simulink model "MIL2"  (R2024b)
settings: Solver=VariableStepAuto  StartTime=0.0  StopTime=0.4  RelTol=1e-3
InitFcn:
  | load('Khinf_QBC_MIL2.mat')
values from neighbouring files (symbols this model uses):
  Ak2 = [0.99999000005 -0.874071604568 92.4139805098 83.0101069502 -184.481272036 -40.5453136884 4.23629025743e-17 -0.390736622587 -19.8991754296 -17.8742726102 39.723699547 8.73047893275 ... (36 elements, 6x6)]    [Khinf_QBC_MIL2.mat]    (also in hinf_discretize_MIL2.m = Kd2.A)
  Bk2 = [0.00079999600002 -0.000349628641827 0.0369655922039 0.0332040427801 -0.0737925088144 -0.0162181254754]    [Khinf_QBC_MIL2.mat]    (also in hinf_discretize_MIL2.m = Kd2.B)
  Ck2 = [17.170141268 -3.69718576515 -0.619129874971 -0.385866142002 -0.162165465963 -0.570961814906]    [Khinf_QBC_MIL2.mat]    (also in hinf_discretize_MIL2.m = Kd2.C)
  Dk2 = 0.00686805650718    [Khinf_QBC_MIL2.mat]    (also in hinf_discretize_MIL2.m = Kd2.D)
  t_vin = 0.2    [mil_metrics2_vin.m]
  Ts2 = 0.0001    [Khinf_QBC_MIL2.mat]    (also in hinf_discretize_MIL2.m = 1/fs)
  Vin_nom = 18    [mil_metrics2_vin.m]
  Vin_step = Vin_nom*(1+vin_pct)    (= 16.2)    [mil_metrics2_vin.m]
undefined symbols (not defined in the file or in its folder): controller_init, D0, dend, DiscIntNeverNeededParam, dspblkCoreblockFVToolHelper, eta, gcbh, Iint_max, K_smc, Ki, Kx, lambda1, numd, phi, Rnom, Tc, Vin, x_op, xi_max
libraries: spsSeriesRLCBranchLib x5, spsCurrentMeasurementLib x3, spsDiodeLib x3, spsVoltageMeasurementLib x3, spsMeanLib x2, spsControlledVoltageSourceLib x1, spsDCVoltageSourceLib x1, slpidlib x1, spsGroundLib x1, spsMosfetLib x1, spsPWMGeneratorDCDCLib x1, sps_lib x1
settings Model: Creator=Asus  LastModifiedBy=yohan
settings ConfigComp: CovMetricSettings=de

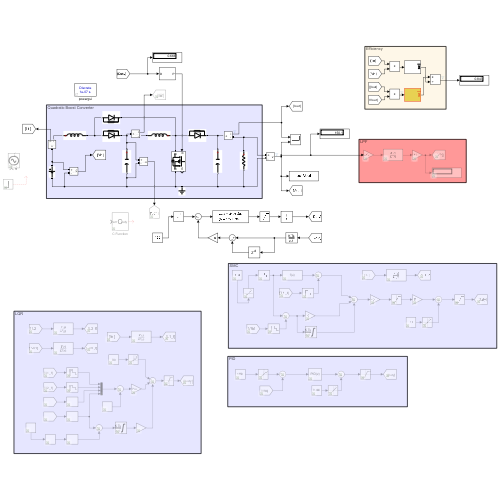
[thumbnail: Simulink's stored preview of the top-level diagram]
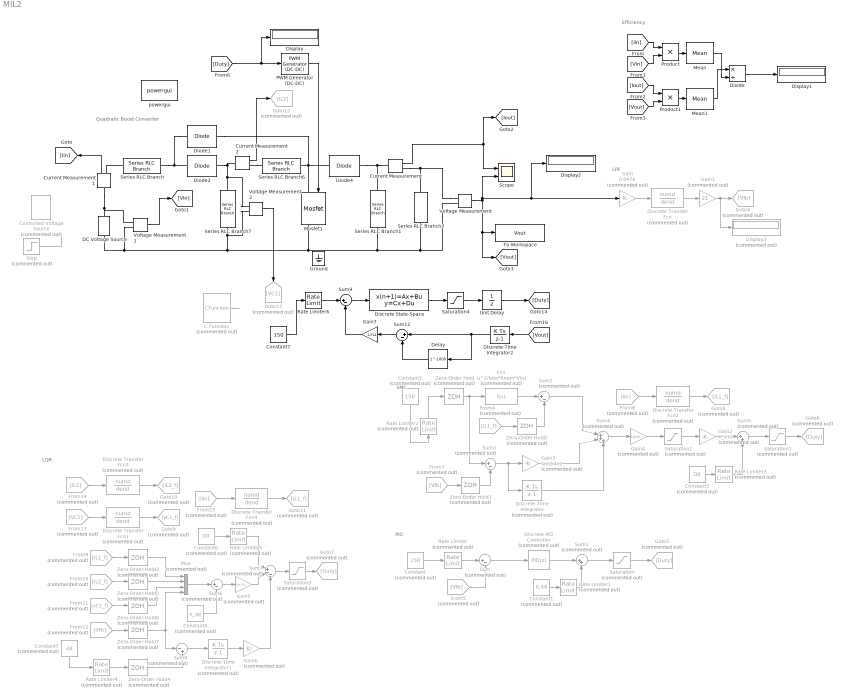
== system MIL2 ==
  note: SMC
  note: LQR
  note: PID
  note: Efficiency
  note: Quadratic Boost Converter
  note: LPF
  C Function : CFunction  Commented=on  OutputCode=duty = controller_step(err, 0.0f);  StartCode=controller_init();  CodegenOutputCode=duty = controller_step(err, 0.0f);  CodegenStartCode=controller_init();  SimCustomHeaderFile=controller_step.h  SimCustomSourceFile=controller_step.c  CustomHeaderFile=controller_step.h  CustomSourceFile=controller_step.c
  Constant : Constant  Commented=on  Value=150
  Constant1 : Constant  Commented=on  Value=0.44
  Constant2 : Constant  Commented=on  Value=150
  Constant3 : Constant  Commented=on  Value=D0
  Constant4 : Constant  Commented=on  Value=x_op
  Constant5 : Constant  Commented=on  Value=48
  Constant6 : Constant  Commented=on  Value=D0
  Constant7 : Constant  Value=150
  Controlled Voltage Source : spsControlledVoltageSourceLib/Controlled Voltage Source  Commented=on  Initialize=on  Source_Type=DC  Amplitude=18  Phase=0  Frequency=0  Measurements=None
  Current Measurement : spsCurrentMeasurementLib/Current Measurement  PhasorSimulation=off  OutputType=Complex  PSBequivalent=0
  Current Measurement1 : spsCurrentMeasurementLib/Current Measurement  PhasorSimulation=off  OutputType=Complex  PSBequivalent=0
  Current Measurement2 : spsCurrentMeasurementLib/Current Measurement  PhasorSimulation=off  OutputType=Complex  PSBequivalent=0
  DC Voltage Source : spsDCVoltageSourceLib/DC Voltage Source  Amplitude=18  Measurements=None
  Delay : Delay  DelayLength=1000  InitialCondition=0  SampleTime=1e-7
  Diode1 : spsDiodeLib/Diode  Ron=0.001  Lon=0  Vf=0  IC=0  UseSnubber=off  Rs=500  Cs=250e-9  Measurements=off
  Diode2 : spsDiodeLib/Diode  Ron=0.001  Lon=0  Vf=0  IC=0  UseSnubber=off  Rs=500  Cs=250e-9  Measurements=off
  Diode4 : spsDiodeLib/Diode  Ron=0.001  Lon=0  Vf=0.8  IC=0  UseSnubber=off  Rs=500  Cs=250e-9  Measurements=off
  Discrete Transfer Fcn{,1..4} (5 alike) : DiscreteTransferFcn  Commented=on  LoadFcn=dspblkCoreblockFVToolHelper(gcbh,'load');  Numerator=numd  Denominator=dend
      settings: CopyFcn=dspblkCoreblockFVToolHelper(gcbh,'copy');  DeleteFcn=dspblkCoreblockFVToolHelper(gcbh,'close');  ModelCloseFcn=dspblkCoreblockFVToolHelper(gcbh,'close');  PreSaveFcn=dspblkCoreblockFVToolHelper(gcbh,'presave');  PostSaveFcn=dspblkCoreblockFVToolHelper(gcbh,'postsave');  CloseFcn=dspblkCoreblockFVToolHelper(gcbh,'close');
  Discrete PID Controller : slpidlib/PID Controller  Commented=on  Controller=PID  Form=Parallel  TimeDomain=Discrete-time  UseExternalTs=off  SampleTime=2e-5  IntegratorMethod=Forward Euler  FilterMethod=Forward Euler  ControllerParametersSource=internal  P=1.0407e-3  I=2.0814e-2  UseKiTs=off  D=2.0814e-6  UseExternalDerivativeSource=off  N=100  UseFilter=on  TunerSelectOption=Transfer Function Based (PID Tuner App)  InitialConditionSource=internal  InitialConditionForIntegrator=0  InitialConditionForFilter=0  DifferentiatorICPrevScaledInput=0  ExternalReset=none  TrackingMode=off  Kt=1  LimitOutput=off  SatLimitsSource=internal  UpperSaturationLimit=inf  LowerSaturationLimit=-inf  LinearizeAsGain=off  AntiWindupMode=none  Kb=1  LimitIntegrator=off  UpperIntegratorSaturationLimit=inf  LowerIntegratorSaturationLimit=-inf  POutMin=[]  POutMax=[]  IOutMin=[]  IOutMax=[]  DOutMin=[]  DOutMax=[]  NOutMin=[]  NOutMax=[]  SumOutMin=[]  SumOutMax=[]  SaturationOutMin=[]  SaturationOutMax=[]  PParamMin=[]  PParamMax=[]  IParamMin=[]  IParamMax=[]  DParamMin=[]  DParamMax=[]  NParamMin=[]  NParamMax=[]  KbParamMin=[]  KbParamMax=[]  KtParamMin=[]  KtParamMax=[]  KbOutMin=[]  KbOutMax=[]  KtOutMin=[]  KtOutMax=[]  IntegratorOutMin=[]  IntegratorOutMax=[]  FilterOutMin=[]  FilterOutMax=[]  SumI1OutMin=[]  SumI1OutMax=[]  SumI2OutMin=[]  SumI2OutMax=[]  SumI3OutMin=[]  SumI3OutMax=[]  SumI4OutMin=[]  SumI4OutMax=[]  SumDOutMin=[]  SumDOutMax=[]  DifferentiatorOutMin=[]  DifferentiatorOutMax=[]  FilterDiffOutCoefMin=[]  FilterDiffOutCoefMax=[]  ReciprocalOutMin=[]  ReciprocalOutMax=[]  SumDenOutMin=[]  SumDenOutMax=[]  SumNumOutMin=[]  SumNumOutMax=[]  DivideOutMin=[]  DivideOutMax=[]  UdiffTsProdOutMin=[]  UdiffTsProdOutMax=[]  NTsProdOutMin=[]  NTsProdOutMax=[]  UintegralTsProdOutMin=[]  UintegralTsProdOutMax=[]  UngainTsProdOutMin=[]  UngainTsProdOutMax=[]  ClampingZeroOutDataTypeStr=Inherit: Inherit via back propagation  ClampingZeroOutMin=[]  ClampingZeroOutMax=[]  FilterDenConstantOutDataTypeStr=Inherit: Inherit via back propagation  FilterDenConstantOutMin=[]  FilterDenConstantOutMax=[]  PCopyOutDataTypeStr=Inherit: Inherit via back propagation  PCopyOutMin=[]  PCopyOutMax=[]  NCopyOutDataTypeStr=Inherit: Inherit via back propagation  NCopyOutMin=[]  NCopyOutMax=[]  IntegratorContinuousStateAttributes=''  IntegratorStateMustResolveToSignalObject=off  IntegratorRTWStateStorageClass=Auto  FilterContinuousStateAttributes=''  FilterStateMustResolveToSignalObject=off  FilterRTWStateStorageClass=Auto  ParallelPVariant=InternalParameters  IdealPVariant=Disabled  IVariant=InternalParameters  DVariant=InternalParameters  IntegratorVariant=Discrete  SatVariant=Disabled  AWVariant=Passthrough  PCopyVariant=Disabled  TRVariant=Disabled  FdbkBlocksVariant=Forward  IdealPFdbkVariant=Disabled  SatFdbkVariant=Disabled  DerivativeFilterVariant=ForwardEulerFilter  NVariant=InternalParameters  NCopyVariant=Disabled  FilterICVariant=InternalICsFilter  IntegratorICVariant=InternalICs  ExternalResetVariant=Disabled  TRSumVariant=Passthrough  SumFdbkVariant=Disabled  SumVariant=Sum_PID  TsampFilterVariant=InternalTs  TsampNgainVariant=Passthrough  TsampIntegralVariant=Disabled_SignalSpec  ExternalSaturationOutDataTypeStr=Inherit: Same as second input  DerivativeSourceVariant=ErrorSignal  PreIntVariant=InternalPreInt
      settings: LibrarySourceBlock=simulink/Discrete/Discrete PID Controller
  Discrete State-Space : DiscreteStateSpace  A=Ak2  B=Bk2  C=Ck2  D=Dk2  SampleTime=Ts2
  Discrete-Time Integrator : DiscreteIntegrator  Commented=on  gainval=lambda2  SampleTime=Tc  LimitOutput=on  UpperSaturationLimit=Iint_max  LowerSaturationLimit=-Iint_max  ICPrevOutput=DiscIntNeverNeededParam  ICPrevScaledInput=DiscIntNeverNeededParam
  Discrete-Time Integrator1 : DiscreteIntegrator  Commented=on  SampleTime=Tc  LimitOutput=on  UpperSaturationLimit=xi_max  LowerSaturationLimit=-xi_max  ICPrevOutput=DiscIntNeverNeededParam  ICPrevScaledInput=DiscIntNeverNeededParam
  Discrete-Time Integrator2 : DiscreteIntegrator  SampleTime=1e-7  ICPrevOutput=DiscIntNeverNeededParam  ICPrevScaledInput=DiscIntNeverNeededParam
  Display : Display
  Display1 : Display
  Display2 : Display
  Display3 : Display  Commented=on
  Divide : Product  Inputs=*/
  Fcn : Fcn  Commented=on  Expr=u^2/(eta*Rnom*Vin)
  From10 : From  Commented=on  GotoTag=iL2_f
  From11 : From  Commented=on  GotoTag=vC1_f
  From12 : From  Commented=on  GotoTag=Vfb
  From13 : From  Commented=on  GotoTag=VC1
  From14 : From  Commented=on  GotoTag=IL2
  From15 : From  Commented=on  GotoTag=Iin
  From4 : From  Commented=on  GotoTag=iL1_f
  From5 : From  Commented=on  GotoTag=Vfb
  From7 : From  Commented=on  GotoTag=Vfb
  From8 : From  Commented=on  GotoTag=Iin
  From9 : From  Commented=on  GotoTag=iL1_f
  Gain : Gain  Commented=on  Gain=0.0476
  Gain1 : Gain  Commented=on  Gain=21
  Gain2 : Gain  Commented=on  Gain=K_smc
  Gain3 : Gain  Commented=on  Gain=lambda1
  Gain4 : Gain  Commented=on  Gain=1/phi
  Gain5 : Gain  Commented=on  Gain=Kx  Multiplication=Matrix(K*u)
  Gain6 : Gain  Commented=on  Gain=Ki
  Gain7 : Gain  Gain=1/Ts2
  Goto10 : Goto  Commented=on  GotoTag=iL2_f
  Goto11 : Goto  Commented=on  GotoTag=iL1_f
  Goto12 : Goto  Commented=on  GotoTag=IL2
  Goto13 : Goto  Commented=on  GotoTag=VC1
  Goto4 : Goto  Commented=on  GotoTag=Vfb
  Goto5 : Goto  Commented=on  GotoTag=Duty
  Goto6 : Goto  Commented=on  GotoTag=Duty
  Goto7 : Goto  Commented=on  GotoTag=Duty
  Goto8 : Goto  Commented=on  GotoTag=iL1_f
  Goto9 : Goto  Commented=on  GotoTag=vC1_f
  Ground : spsGroundLib/Ground  LConnTagsString=a
  Mean : spsMeanLib/Mean  Freq=1000  Vinit=0  Ts=0
  Mean1 : spsMeanLib/Mean  Freq=1000  Vinit=0  Ts=0
  Mosfet1 : spsMosfetLib/Mosfet  Ron=0.1  Lon=0  Rd=0.01  Vfd=0  IC=0  Rs=1e5  Cs=inf  Measurements=on
  Mux : Mux  Commented=on
  PWM Generator (DC-DC) : spsPWMGeneratorDCDCLib/PWM Generator (DC-DC)  Fsw=10000  Ts=0
  Product : Product
  Product1 : Product
  Rate Limiter : RateLimiter  Commented=on  RisingSlewLimit=1600  SampleTimeMode=inherited
  Rate Limiter1 : RateLimiter  Commented=on  RisingSlewLimit=15  SampleTimeMode=inherited
  Rate Limiter2 : RateLimiter  Commented=on  RisingSlewLimit=1600  FallingSlewLimit=-inf  SampleTimeMode=inherited
  Rate Limiter3 : RateLimiter  Commented=on  RisingSlewLimit=15  FallingSlewLimit=-inf  SampleTimeMode=inherited
  Rate Limiter4 : RateLimiter  Commented=on  RisingSlewLimit=1600  FallingSlewLimit=-inf  SampleTimeMode=inherited
  Rate Limiter5 : RateLimiter  Commented=on  RisingSlewLimit=15  FallingSlewLimit=-inf  SampleTimeMode=inherited
  Rate Limiter6 : RateLimiter  RisingSlewLimit=150/0.025  FallingSlewLimit=-150/0.025  SampleTimeMode=inherited
  Saturation : Saturate  Commented=on  UpperLimit=0.8  LowerLimit=0
  Saturation1 : Saturate  Commented=on  UpperLimit=0.6  LowerLimit=0
  Saturation2 : Saturate  Commented=on  UpperLimit=1  LowerLimit=-1
  Saturation3 : Saturate  Commented=on  UpperLimit=0.6  LowerLimit=0
  Saturation4 : Saturate  UpperLimit=5  LowerLimit=-5
  Scope : Scope  NumInputPorts=2
      settings: InitFcn=load('Khinf_QBC_MIL1.mat')  OpenFcn=load('Khinf_QBC_MIL1.mat')
  Series RLC Branch : spsSeriesRLCBranchLib/Series RLC Branch  LConnTagsString=__new0  RConnTagsString=__new0  BranchType=L  Resistance=0.005  Inductance=0.001  SetiL0=off  InitialCurrent=0  Capacitance=1e-6  Setx0=off  InitialVoltage=0  Measurements=None
  Series RLC Branch1 : spsSeriesRLCBranchLib/Series RLC Branch  LConnTagsString=__new0  RConnTagsString=__new0  BranchType=C  Resistance=0.01  Inductance=1e-3  SetiL0=off  InitialCurrent=0  Capacitance=0.0001  Setx0=off  InitialVoltage=0  Measurements=None
  Series RLC Branch2 : spsSeriesRLCBranchLib/Series RLC Branch  LConnTagsString=__new0  RConnTagsString=__new0  BranchType=R  Resistance=135  Inductance=1e-3  SetiL0=off  InitialCurrent=0  Capacitance=1e-6  Setx0=off  InitialVoltage=0  Measurements=Branch voltage and current
  Series RLC Branch6 : spsSeriesRLCBranchLib/Series RLC Branch  LConnTagsString=__new0  RConnTagsString=__new0  BranchType=L  Resistance=0.01  Inductance=0.003  SetiL0=off  InitialCurrent=0  Capacitance=1.2e-6  Setx0=off  InitialVoltage=0  Measurements=None
  Series RLC Branch7 : spsSeriesRLCBranchLib/Series RLC Branch  LConnTagsString=__new0  RConnTagsString=__new0  BranchType=C  Resistance=0.01  Inductance=1e-3  SetiL0=off  InitialCurrent=0  Capacitance=0.0001  Setx0=off  InitialVoltage=0  Measurements=None
  Step : Step  Commented=on  Time=t_vin  Before=Vin_nom  After=Vin_step  SampleTime=0
  Sum{,2..3,6} (4 alike) : Sum  Commented=on  Inputs=|+-
  Sum1 : Sum  Commented=on  Inputs=|++
  Sum12 : Sum  Inputs=|+-
  Sum4 : Sum  Commented=on  Inputs=|+++
  Sum5 : Sum  Commented=on  Inputs=|++
  Sum7 : Sum  Commented=on  Inputs=|+--
  Sum8 : Sum  Commented=on  Inputs=|-+
  Sum9 : Sum  Inputs=|+-
  To Workspace : ToWorkspace  VariableName=Vout  SaveFormat=Timeseries  SampleTime=-1
  Unit Delay : UnitDelay  SampleTime=Ts2
  Voltage Measurement : spsVoltageMeasurementLib/Voltage Measurement  PhasorSimulation=off  OutputType=Complex  PSBequivalent=0
  Voltage Measurement1 : spsVoltageMeasurementLib/Voltage Measurement  PhasorSimulation=off  OutputType=Complex  PSBequivalent=0
  Voltage Measurement2 : spsVoltageMeasurementLib/Voltage Measurement  PhasorSimulation=off  OutputType=Complex  PSBequivalent=0
  Zero-Order Hold{,1..7} (8 alike) : ZeroOrderHold  Commented=on  SampleTime=Tc
  powergui : sps_lib/powergui  Priority=1  SimulationMode=Discrete  SampleTime=1e-7  frequency=60  Iterations=50  frequencyindice=0  Pbase=100e6  ErrMax=1e-4  UnitsV=kV  UnitsW=MW  buscounter=0  FunctionMessages=off  echomessages=off  EnableUseOfTLC=off  CurrentSourceSwitches=off  DisableSnubberDevices=off  DisableRonSwitches=off  DisableVfSwitches=off  DisplayEquations=off  AutomaticDiscreteSolvers=off  SolverType=Backward Euler  Interpol=off  ExternalGateDelay=off  methode=off  Ts=10  x0status=blocks  SPID=off  SwTol=0  HookPort=off  NonlinearTolerance=1e-4  nMaxIteration=100  ContinueOnMaxIteration=off  RestoreLinks=warning  ResistiveCurrentMeasurement=off  Frange=[0:2:500]  Ylog=off  Xlog=on  ShowGrid=off  save=off  variable=ZData  structure=0  ZoomFFT=off  StartTime=0.0  cycles=1  DisplayStyle=1  fundamental=60  FreqAxis=off  MaxFrequency=1000  frequencyindicesteady=1  RmsSteady=1  display=off
  wires:
  Constant7/1 -> Rate Limiter6/1
  Constant4/1 -> Sum6/2
  Discrete Transfer Fcn4/1 -> Goto11/1
  Constant2/1 -> Rate Limiter2/1
  Mux/1 -> Sum6/1
  Divide/1 -> Display1/1
  Constant1/1 -> Rate Limiter1/1
  Gain2/1 -> Sum5/1
  Sum6/1 -> Gain5/1
  Voltage Measurement/1 -> Gain/1, Display2/1, Scope/2, To Workspace/1, [Vout]
  From12/1 -> Zero-Order Hold7/1
  Discrete Transfer Fcn3/1 -> Goto10/1
  Gain5/1 -> Sum7/2
  Voltage Measurement2/1 -> Goto13/1
  Gain3/1 -> Sum4/2
  Zero-Order Hold3/1 -> Mux/1
  Fcn/1 -> Sum2/1
  Rate Limiter3/1 -> Sum5/2
  Zero-Order Hold2/1 -> Sum2/2
  From8/1 -> Discrete Transfer Fcn2/1
  Rate Limiter1/1 -> Sum1/2
  Saturation3/1 -> Goto7/1
  Constant6/1 -> Rate Limiter5/1
  From9/1 -> Zero-Order Hold3/1
  Rate Limiter2/1 -> Zero-Order Hold/1
  Sum3/1 -> Discrete-Time Integrator/1, Gain3/1
  Mean1/1 -> Divide/1
  Sum4/1 -> Gain4/1
  [Vin] -> Product/2
  Product/1 -> Mean/1
  Constant5/1 -> Rate Limiter4/1
  Sum7/1 -> Saturation3/1
  From15/1 -> Discrete Transfer Fcn4/1
  From11/1 -> Zero-Order Hold6/1
  Sum8/1 -> Discrete-Time Integrator1/1
  From10/1 -> Zero-Order Hold5/1
  Saturation2/1 -> Gain2/1
  Sum5/1 -> Saturation1/1
  Constant3/1 -> Rate Limiter3/1
  PWM Generator (DC-DC)/1 -> Mosfet1/1
  Rate Limiter4/1 -> Zero-Order Hold4/1
  Mean/1 -> Divide/2
  Rate Limiter/1 -> Sum/1
  Discrete-Time Integrator1/1 -> Gain6/1
  Voltage Measurement1/1 -> [Vin]
  Sum/1 -> Discrete PID Controller/1
  From14/1 -> Discrete Transfer Fcn3/1
  Discrete Transfer Fcn2/1 -> Goto8/1
  Current Measurement/1 -> [Iout], Scope/1
  Gain6/1 -> Sum7/3
  Gain4/1 -> Saturation2/1
  [Iout] -> Product1/1
  Gain/1 -> Discrete Transfer Fcn/1
  Zero-Order Hold4/1 -> Sum8/2
  Sum1/1 -> Saturation/1
  From4/1 -> Zero-Order Hold2/1
  Zero-Order Hold6/1 -> Mux/3
  Product1/1 -> Mean1/1
  From5/1 -> Sum/2
  Zero-Order Hold/1 -> Fcn/1, Sum3/1
  Discrete Transfer Fcn/1 -> Gain1/1
  Discrete PID Controller/1 -> Sum1/1
  Current Measurement2/1 -> Goto12/1
  [Duty] -> Display/1, PWM Generator (DC-DC)/1
  Discrete-Time Integrator/1 -> Sum4/3
  Discrete Transfer Fcn1/1 -> Goto9/1
  Rate Limiter5/1 -> Sum7/1
  Zero-Order Hold7/1 -> Sum8/1, Mux/4
  Current Measurement1/1 -> [Iin]
  Saturation1/1 -> Goto6/1
  [Iin] -> Product/1
  [Vout] -> Product1/2
  From7/1 -> Zero-Order Hold1/1
  From13/1 -> Discrete Transfer Fcn1/1
  Zero-Order Hold5/1 -> Mux/2
  Saturation/1 -> Goto5/1
  Constant/1 -> Rate Limiter/1
  Sum2/1 -> Sum4/1
  Zero-Order Hold1/1 -> Sum3/2
  Gain1/1 -> Display3/1, Goto4/1
  Unit Delay/1 -> [Duty]
  Saturation4/1 -> Unit Delay/1
  Rate Limiter6/1 -> Sum9/1
  Sum12/1 -> Gain7/1
  Delay/1 -> Sum12/2
  Gain7/1 -> Sum9/2
  Discrete-Time Integrator2/1 -> Sum12/1, Delay/1
  [Vout] -> Discrete-Time Integrator2/1
  Step/1 -> ?
  C Function/1 -> ?
  Sum9/1 -> Discrete State-Space/1
  Discrete State-Space/1 -> Saturation4/1
  connections:
  Diode2/RConn1 -- Series RLC Branch7/LConn1 -- Voltage Measurement2/LConn1 -- Current Measurement2/LConn1
  Voltage Measurement/LConn1 -- Series RLC Branch2/LConn1 -- Current Measurement/RConn1
  Diode1/LConn1 -- Diode2/LConn1 -- Series RLC Branch/RConn1
  Current Measurement/LConn1 -- Diode4/RConn1 -- Series RLC Branch1/LConn1
  Series RLC Branch7/RConn1 -- DC Voltage Source/LConn1 -- Voltage Measurement1/LConn2 -- Series RLC Branch2/RConn1 -- Voltage Measurement/LConn2 -- Series RLC Branch1/RConn1 -- Mosfet1/RConn1 -- Voltage Measurement2/LConn2
  Voltage Measurement1/LConn1 -- DC Voltage Source/RConn1 -- Current Measurement1/LConn1
  Diode1/RConn1 -- Mosfet1/LConn1 -- Series RLC Branch6/LConn1 -- Diode4/LConn1
  Current Measurement2/RConn1 -- Series RLC Branch6/RConn1
  Current Measurement1/RConn1 -- Series RLC Branch/LConn1
